simulink model "printable_simulation"  (R2024b)
settings: Solver=ode1be  StartTime=0.0  StopTime=10  FixedStep=0.001  RelTol=1e-3
model workspace (MAT data in the model file):
  AMP = 1
  FREQ = 1
  i_abc = 1
undefined symbols (not defined in the file or in its folder): Drive_wheel, Driveshaft, eff_shaft, f_OVD, i, J_S21, Jr2, K, M_curve_1, M_curve_2, M_total, mi_c, mi_s, Mode, N_clutch, n_curve_1, n_curve_2, n_max_1, n_max_2, n_surfaces, Pl, r_eq_clutch, r_geom, Shaft, sigma0, sigma1, sigma2, Spurs_Inertia, Stage1, Stage2, Stage3, vs, wheel_width
libraries: simulink x12, slpidlib x1
(part 3 of 3)

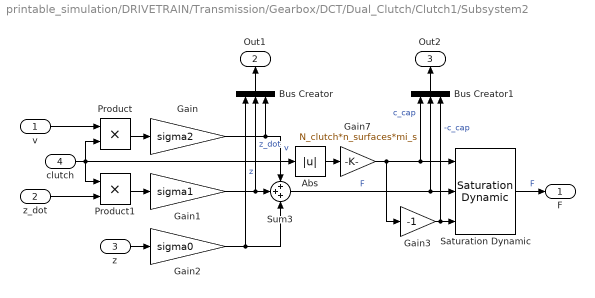
== system printable_simulation/DRIVETRAIN/Transmission/Gearbox/DCT/Dual_Clutch/Clutch1/Subsystem2 ==
  v : Inport
  z_dot : Inport  Port=2
  z : Inport  Port=3
  clutch : Inport  Port=4
  Abs : Abs  SaturateOnIntegerOverflow=off
  Bus Creator : BusCreator  Inputs=3
  Bus Creator1 : BusCreator  Inputs=3
  Gain : Gain  Gain=sigma2
  Gain1 : Gain  Gain=sigma1
  Gain2 : Gain  Gain=sigma0
  Gain3 : Gain  Gain=-1
  Gain7 : Gain  Gain=N_clutch*n_surfaces*mi_s
  Product : Product
  Product1 : Product
  Saturation Dynamic : simulink/Discontinuities/Saturation Dynamic  OutMin=[]  OutMax=[]  OutDataTypeStr=Inherit: Same as second input  OutDataType=fixdt(1, 16)  OutScaling=2^-10  DoSatur=off
  Sum3 : Sum  Inputs=+++
  F : Outport
  Out1 : Outport  Port=2
  Out2 : Outport  Port=3
  wires:
  Product/1 -> Gain/1
  Bus Creator/1 -> Out1/1
  z/1 -> Gain2/1
  z_dot/1 -> Product1/2
  Gain1/1 -> Bus Creator/2, Sum3/2  "z_dot"
  Saturation Dynamic/1 -> F/1  "F"
  Gain2/1 -> Bus Creator/1, Sum3/3  "z"
  Gain/1 -> Sum3/1, Bus Creator/3  "v"
  v/1 -> Product/1
  clutch/1 -> Product1/1, Abs/1, Product/2
  Product1/1 -> Gain1/1
  Abs/1 -> Gain7/1
  Gain7/1 -> Bus Creator1/1, Saturation Dynamic/1, Gain3/1  "c_cap"
  Gain3/1 -> Bus Creator1/3, Saturation Dynamic/3  "-c_cap"
  Sum3/1 -> Bus Creator1/2, Saturation Dynamic/2  "F"
  Bus Creator1/1 -> Out2/1

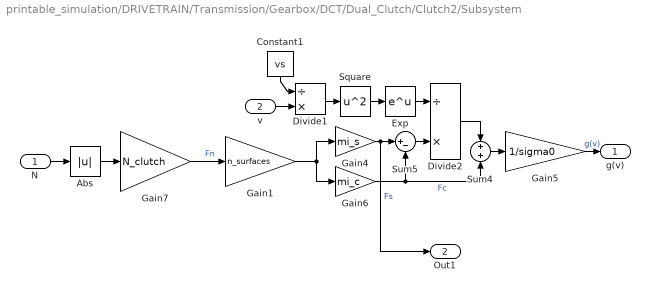
== system printable_simulation/DRIVETRAIN/Transmission/Gearbox/DCT/Dual_Clutch/Clutch2/Subsystem ==
  N : Inport
  v : Inport  Port=2
  Abs : Abs  SaturateOnIntegerOverflow=off
  Constant1 : Constant  Value=vs
  Divide1 : Product  Inputs=/*
  Divide2 : Product  Inputs=/*
  Exp : Math
  Gain1 : Gain  Gain=n_surfaces
  Gain4 : Gain  Gain=mi_s
  Gain5 : Gain  Gain=1/sigma0
  Gain6 : Gain  Gain=mi_c
  Gain7 : Gain  Gain=N_clutch
  Square : Math  Operator=square
  Sum4 : Sum  Inputs=+|+
  Sum5 : Sum  Inputs=|+-
  g(v) : Outport
  Out1 : Outport  Port=2
  wires:
  Gain1/1 -> Gain6/1, Gain4/1
  Gain4/1 -> Out1/1, Sum5/1  "Fs"
  Abs/1 -> Gain7/1
  v/1 -> Divide1/2
  N/1 -> Abs/1
  Gain5/1 -> g(v)/1  "g(v)"
  Square/1 -> Exp/1
  Divide1/1 -> Square/1
  Constant1/1 -> Divide1/1
  Gain7/1 -> Gain1/1  "Fn"
  Exp/1 -> Divide2/1
  Gain6/1 -> Sum5/2, Sum4/2  "Fc"
  Divide2/1 -> Sum4/1
  Sum5/1 -> Divide2/2
  Sum4/1 -> Gain5/1

== system printable_simulation/DRIVETRAIN/Transmission/Gearbox/DCT/Dual_Clutch/Clutch2/Subsystem1 ==
  v : Inport
  g(v) : Inport  Port=2
  "clutch " : Inport  Port=3
  Abs1 : Abs  SaturateOnIntegerOverflow=off
  Compare To Constant : simulink/Logic and Bit Operations/Compare To Constant  relop=<=  const=0.001  OutDataTypeStr=boolean
  Divide : Product  Inputs=*/
  Integrator : Integrator  ExternalReset=level
  Product2 : Product
  Saturation : Saturate  UpperLimit=inf  LowerLimit=0.000001
  Scope : Scope  NumInputPorts=2
  Sum2 : Sum  Inputs=|+-
  z_dot : Outport
  z : Outport  Port=2
  wires:
  Compare To Constant/1 -> Integrator/2
  g(v)/1 -> Saturation/1, Scope/2
  Product2/1 -> Sum2/2
  Abs1/1 -> Divide/1
  Saturation/1 -> Divide/2, Scope/1
  Sum2/1 -> z_dot/1, Integrator/1  "z_dot"
  v/1 -> Sum2/1, Abs1/1
  Divide/1 -> Product2/1
  Integrator/1 -> z/1, Product2/2  "z"
  "clutch "/1 -> Compare To Constant/1

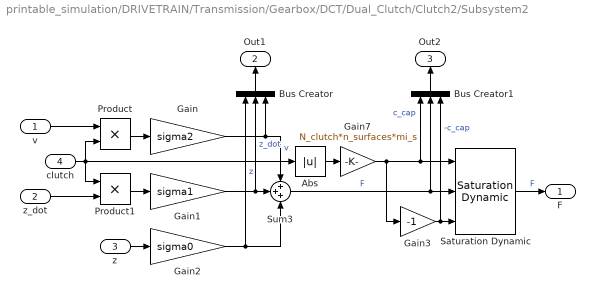
== system printable_simulation/DRIVETRAIN/Transmission/Gearbox/DCT/Dual_Clutch/Clutch2/Subsystem2 ==
  v : Inport
  z_dot : Inport  Port=2
  z : Inport  Port=3
  clutch : Inport  Port=4
  Abs : Abs  SaturateOnIntegerOverflow=off
  Bus Creator : BusCreator  Inputs=3
  Bus Creator1 : BusCreator  Inputs=3
  Gain : Gain  Gain=sigma2
  Gain1 : Gain  Gain=sigma1
  Gain2 : Gain  Gain=sigma0
  Gain3 : Gain  Gain=-1
  Gain7 : Gain  Gain=N_clutch*n_surfaces*mi_s
  Product : Product
  Product1 : Product
  Saturation Dynamic : simulink/Discontinuities/Saturation Dynamic  OutMin=[]  OutMax=[]  OutDataTypeStr=Inherit: Same as second input  OutDataType=fixdt(1, 16)  OutScaling=2^-10  DoSatur=off
  Sum3 : Sum  Inputs=+++
  F : Outport
  Out1 : Outport  Port=2
  Out2 : Outport  Port=3
  wires:
  Product/1 -> Gain/1
  Bus Creator/1 -> Out1/1
  z/1 -> Gain2/1
  z_dot/1 -> Product1/2
  Gain1/1 -> Bus Creator/2, Sum3/2  "z_dot"
  Saturation Dynamic/1 -> F/1  "F"
  Gain2/1 -> Bus Creator/1, Sum3/3  "z"
  Gain/1 -> Sum3/1, Bus Creator/3  "v"
  v/1 -> Product/1
  clutch/1 -> Product1/1, Abs/1, Product/2
  Product1/1 -> Gain1/1
  Abs/1 -> Gain7/1
  Gain7/1 -> Bus Creator1/1, Saturation Dynamic/1, Gain3/1  "c_cap"
  Gain3/1 -> Bus Creator1/3, Saturation Dynamic/3  "-c_cap"
  Sum3/1 -> Bus Creator1/2, Saturation Dynamic/2  "F"
  Bus Creator1/1 -> Out2/1

== system printable_simulation/DRIVETRAIN/Transmission/Gearbox/DCT/Stage_2.1/Spur/Spur2 ==
  Torque_in : Inport
  Speed_fdbk : Inport  Port=2
  Derivative1 : Derivative
  Gain : Gain  Gain=i
  Gain3 : Gain  Gain=J2
  Gain4 : Gain  Gain=i
  Sum1 : Sum  Inputs=|+-
  Torque_out : Outport
  phi_dot : Outport  Port=2
  wires:
  Sum1/1 -> Torque_out/1
  Gain3/1 -> Sum1/2
  Torque_in/1 -> Gain/1
  Speed_fdbk/1 -> Derivative1/1, Gain4/1
  Derivative1/1 -> Gain3/1
  Gain4/1 -> phi_dot/1
  Gain/1 -> Sum1/1

== system printable_simulation/DRIVETRAIN/Transmission/Gearbox/DCT/Stage_2.2/Spur/Spur2 ==
  Torque_in : Inport
  Speed_fdbk : Inport  Port=2
  Derivative1 : Derivative
  Gain : Gain  Gain=i
  Gain3 : Gain  Gain=J2
  Gain4 : Gain  Gain=i
  Sum1 : Sum  Inputs=|+-
  Torque_out : Outport
  phi_dot : Outport  Port=2
  wires:
  Sum1/1 -> Torque_out/1
  Torque_in/1 -> Gain/1
  Speed_fdbk/1 -> Derivative1/1, Gain4/1
  Derivative1/1 -> Gain3/1
  Gain3/1 -> Sum1/2
  Gain/1 -> Sum1/1
  Gain4/1 -> phi_dot/1

== system printable_simulation/DRIVETRAIN/Transmission/Gearbox/DCT/Stage_3/Spur/Shaft ==
  Torque_in : Inport
  Speed_fdbk : Inport  Port=2
  Derivative : Derivative
  Gain3 : Gain  Gain=J
  Sum1 : Sum  Inputs=|+-
  Torque_out : Outport
  phi_dot : Outport  Port=2
  wires:
  Speed_fdbk/1 -> phi_dot/1, Derivative/1
  Sum1/1 -> Torque_out/1
  Derivative/1 -> Gain3/1
  Torque_in/1 -> Sum1/1
  Gain3/1 -> Sum1/2

== system printable_simulation/DRIVETRAIN/Transmission/Gearbox/DCT/Stage_3/Spur/Spur3 ==
  Torque_in : Inport
  Speed_fdbk : Inport  Port=2
  Derivative : Derivative
  Derivative1 : Derivative
  Gain1 : Gain  Gain=i
  Gain2 : Gain  Gain=J2
  Gain3 : Gain  Gain=J1
  Gain5 : Gain  Gain=i
  Sum1 : Sum  Inputs=|+-
  Sum2 : Sum  Inputs=|+-
  Torque_out : Outport
  phi_dot : Outport  Port=2
  wires:
  Sum2/1 -> Torque_out/1
  Torque_in/1 -> Sum1/1
  Gain1/1 -> Sum2/1
  Sum1/1 -> Gain1/1
  Speed_fdbk/1 -> Gain5/1, Derivative/1
  Gain5/1 -> phi_dot/1, Derivative1/1
  Derivative/1 -> Gain2/1
  Derivative1/1 -> Gain3/1
  Gain3/1 -> Sum1/2
  Gain2/1 -> Sum2/2

== stateflow chart printable_simulation/CONTROLS/MCU/AMT ==
  state Steady_State_G1
  state Taking_Off
  state Torque_Blend_PH1
  state Torque_Blend_PH5
  state Steady_State_G2
  state DecoupleStage_PH2
  state ShiftingStage_PH4
  state Synch_PH3
  state15 -> state18 [order 1] : [n_engine > n_upshift]
  state35 -> state15 [order 2] : [GearSet==1]
  state15 -> state5 [order 2] : [Speed == 0]
  state5 -> state15 : [n_engine > 100]
  (default) -> state5
  state20 -> state5 [order 2] : [Speed == 0]
  state20 -> state18 [order 1] : [n_engine < n_downshift]
  state35 -> state20 [order 1] : [GearSet == 2]
  state18 -> state19
  state44 -> state35
  state19 -> state26
  state26 -> state44
  data: output; input; input; output

== stateflow chart printable_simulation/CONTROLS/MCU/DCT_MCU ==
  state Steady_State_G1
  state Torque_Phase1
  state Inertia_phase2
  state Taking_Off
  state Inertia_phase1
  state Torque_Phase2
  state Steady_State_G2
  state259 -> state291 [order 2] : [n_engine > n_upshift]
  state255 -> state259 : [delta_w2 == 0]
  state259 -> state268 [order 1] : [Speed == 0]
  state268 -> state259 : [M_MCU >= M_EM_Driver]
  state291 -> state292 : [M_clutch1 <= 0]
  state260 -> state255 : [M_clutch2 <=0]
  (default) -> state268
  state269 -> state268 [order 2] : [Speed == 0]
  state269 -> state260 [order 1] : [n_engine < n_downshift]
  state292 -> state269 : [delta_w1 == 0]
  data: M_MCU output =0; w_m input; M_EM_Driver input; C2_set output =1; Gear input double size=1; M_m input; M_c1 input; M_c2 input; Pedal input; Take_off output =0; shifting_stage output =0; clutch1Set output =1; clutch2Set output =0; GearSet output int32 =1; st input; M_shift local; w_spur21 input; tshift input; i1 input; i2 input; time input; w_spur11 input; t local double size=1 =0; TO_t input; delta_w local =0; u local; w_shift input; reset local =0; s local; t0 local; w_ref local; c2 local; c1 local; M_ref local; M2_ref local; M_inertia local; delta_M local; w_t output; M_t output =0; e local; t1 local; w_start local; M_i local =0; bt input; s1 local

== stateflow chart printable_simulation/CONTROLS/MCU/TDT ==
  state Steady_State_G1
  state Taking_Off
  state Torque_Blend_PH1
  state Torque_Blend_PH7
  state Steady_State_G2
  state Torque_Blend_PH2
  state Torque_Blend_PH6
  state Neutral_Stage_PH3
  state Synch_PH4
  state UpDownshift_PH5
  state15 -> state18 [order 1] : [n_engine > n_upshift]
  state35 -> state15 [order 2] : [GearSet==1]
  state15 -> state5 [order 2] : [Speed == 0]
  state5 -> state15 : [M_MCU >= M_EM_Driver]
  (default) -> state5
  state20 -> state5 [order 2] : [Speed == 0]
  state20 -> state18 [order 1] : [n_engine < n_downshift]
  state35 -> state20 [order 1] : [GearSet == 2]
  state18 -> state19
  state33 -> state35
  state19 -> state24
  state31 -> state33
  state24 -> state26
  state26 -> state31
  data: output; input; input; output; n_engine input; GearSet input; Speed input; M_EM_Driver input; n_upshift input; n_downshift input; M_MCU parameter
